simulink model "Thesis"  (Simulink 7.3)
settings: Solver=FixedStepDiscrete  SolverMode=SingleTasking  StartTime=0.0  StopTime=inf  FixedStep=1e-6  RelTol=1e-3
libraries: dsPICdrivers x7, simulink x3
settings Model: Creator=Administrateur  LastModifiedBy=Saeed
settings OptimizationCC: InlineParams=on  InitFltsAndDblsToZero=on  OptimizeModelRefInitCode=on  LifeSpan=1
settings DebuggingCC: SaveWithParameterizedLinksMsg=none
settings HardwareCC: ProdBitPerInt=16  ProdEndianess=LittleEndian  ProdWordSize=16  ProdHWDeviceType=16-bit Generic
settings RTWCC: SystemTargetFile=dspic.tlc  MakeCommand=make_CreateMPLAB  TemplateMakefile=dspic_pic30_gcc.tmf  PostCodeGenCommand=dsPIC_Compile()  Description=Embedded Target for Microchip dsPIC (real-time)  ProcessScript=dspic_make_rtw_hook
settings CodeAppCC: IgnoreCustomStorageClasses=off
settings STFCustomTargetCC: TargetFcnLib=ansi_tfl_tmw.mat  IncludeMdlTerminateFcn=off  CombineOutputUpdateFcns=on  ERTCustomFileBanners=on  SupportNonFinite=off  SupportComplex=off  SupportNonInlinedSFcns=off  CPPClassGenCompliant=on  SystemTargetFile=dspic.tlc
settings ERTTargetCC: TargetFcnLib=ansi_tfl_tmw.mat  MultiwordLength=2048  ParMdlRefBuildCompliant=off  CompOptLevelCompliant=off  IncludeMdlTerminateFcn=off  ERTFirstTimeCompliant=off  SupportNonFinite=off  SupportComplex=off  SupportContinuousTime=on  ModelStepFunctionPrototypeControlCompliant=off  ExtModeMexFile=ext_serial_win32_comm  InlinedParameterPlacement=NonHierarchical  ERTSrcFileBannerTemplate=dsPIC_code_template.cgt  ERTHdrFileBannerTemplate=dsPIC_code_template.cgt  ERTDataSrcFileTemplate=dsPIC_code_template.cgt  ERTDataHdrFileTemplate=dsPIC_code_template.cgt  ERTCustomFileTemplate=dsPIC_main.tlc
settings CustomProperty: DataType=string  Value=E:\PROGRA~1\MATLAB\R2009a\bin\win32\gmake

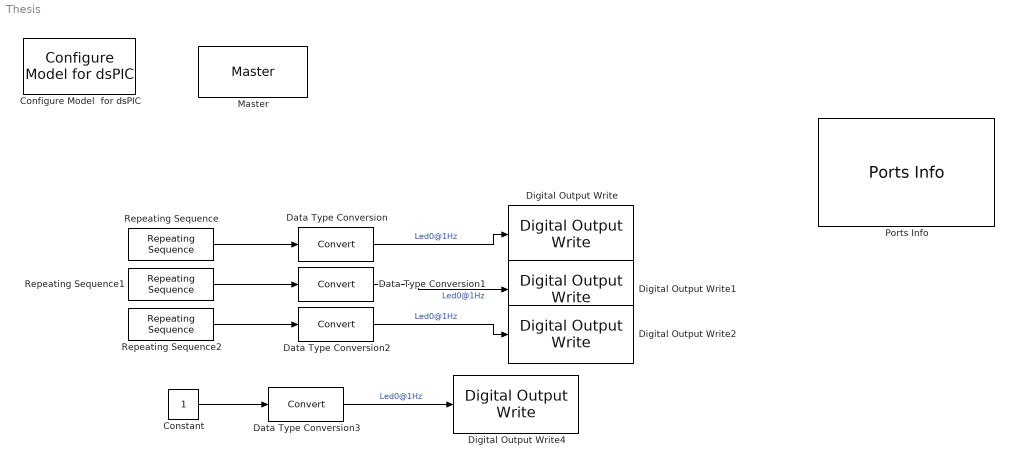
== system Thesis ==
  Configure Model  for dsPIC : dsPICdrivers/Simulink Configuration/Configure Model  for dsPIC
  Constant : Constant  OutDataType=fixdt(1, 16)  OutScaling=2^0  SampleTime=-1
  Data Type Conversion{,1..3} (4 alike) : DataTypeConversion  OutDataType=fixdt(0,8,4)  RndMeth=Nearest
  Digital Output Write : dsPICdrivers/Digital I//O/Digital Output Write  Tag=dsPIC_Digital_Output  Priority=5  PORT=F  Pin=[1]  Simultaneous=off  OrderingInOutPopup=None
  Digital Output Write1 : dsPICdrivers/Digital I//O/Digital Output Write  Tag=dsPIC_Digital_Output  Priority=5  PORT=F  Pin=[2]  Simultaneous=off  OrderingInOutPopup=None
  Digital Output Write2 : dsPICdrivers/Digital I//O/Digital Output Write  Tag=dsPIC_Digital_Output  Priority=5  PORT=G  Pin=[1]  Simultaneous=off  OrderingInOutPopup=None
  Digital Output Write4 : dsPICdrivers/Digital I//O/Digital Output Write  Tag=dsPIC_Digital_Output  Priority=5  PORT=A  Pin=[5]  Simultaneous=off  OrderingInOutPopup=None
  Master : dsPICdrivers/Master  Tag=dsPIC_MASTER  Priority=1  TimeStepType=Free Run  picType=33fJ256MC710a  fcy=4000000  Quartz_33f=8e6  PLLActive_33f=off  fcyDesired_33f=4000000  tmr1="[1  5  4]"  tmr1Info="Time Step : 1e-006  ;   Error : 0%  PR1=3"  tmr2345="[0  0  0  0  0  0  0  0]"  tmr2345cfg=[-1 -1 -1 -1 -1 -1 -1 -1]  IOautoConf=on  typePort="[ 0   0   0   0   0  10   0   0   0   0   0   0   0   0   0   0   0   0   0   0   0   0   0   0   0   0   0   0   0   0   0   0   0   0   0   0   0   0   0   0   0   0   0   0   0   0   0   0   0   0   0   0   0   0   0   0   0   0   0   0   0   0   0   0   0   0   0   0   0   0   0   0   0   0   0   0   0   0   0   0   0  10  10   0   0   0   0   0   0   0   0   0   0   0   0   0   0  10   0   0   0   0   0   0   0   0   0   0   0   0   0   0 ]"  TRIS="[ 65503  65535  65535  65535  65535  65529  65533 ]"  ADPCFG=0  MasterBusyPort=None  MasterOverloadPort=None  FOSC=Quartz (XT - HS)  ClockSwitchMonitor=Both disabled  TempProtection_33f=TEMP_ON  FPBOR=<empty>  PWRT=disable  MCLR=<empty>  ICD=ICS_PGD1  JTAGEN=JTAGEN_OFF  PowerSave=off  OverrideFcy=off  NewFcy=1e6  PR2345="[65535  65535  65535  65535  65535  65535  65535  65535]"
  Ports Info : dsPICdrivers/Ports Info  Tag=dsPIC_PortInfo
  Repeating Sequence : simulink/Sources/Repeating Sequence  SystemSampleTime=-1  rep_seq_t=[0 0 .2 .2 1]*(1/30e3)  rep_seq_y=[0 1 1 0 0]
  Repeating Sequence1 : simulink/Sources/Repeating Sequence  SystemSampleTime=-1  rep_seq_t=[0 0.4 .4 .6 .6 1]*(1/30e3)  rep_seq_y=[0 0 1 1 0 0]
  Repeating Sequence2 : simulink/Sources/Repeating Sequence  SystemSampleTime=-1  rep_seq_t=[0 .7 .7 .9 .9 1]*(1/30e3)  rep_seq_y=[0 0 1 1 0 0]
  wires:
  Repeating Sequence2/1 -> Data Type Conversion2/1
  Data Type Conversion2/1 -> Digital Output Write2/1  "Led0@1Hz"
  Constant/1 -> Data Type Conversion3/1
  Data Type Conversion3/1 -> Digital Output Write4/1  "Led0@1Hz"
  Data Type Conversion/1 -> Digital Output Write/1  "Led0@1Hz"
  Repeating Sequence/1 -> Data Type Conversion/1
  Repeating Sequence1/1 -> Data Type Conversion1/1
  Data Type Conversion1/1 -> Digital Output Write1/1  "Led0@1Hz"
